simulink model "ZT_VehCtrl_18B_CAN"  (R2018b)
settings: Solver=FixedStepAuto  StartTime=0.0  StopTime=inf  FixedStep=0.005  RelTol=1e-3
InitFcn:
  | mbd_mpc_consistency_checks(bdroot(gcs));
values from neighbouring files (symbols this model uses):
  BatoverTempTh = single(80)    [VCU_INIT.m]
  BRS_PwrValid = single(5)    [VCU_INIT.m]
  BRSEnSpdTh1 = single(10)    [VCU_INIT.m]
  BRSEnSpdTh2 = single(20)    [VCU_INIT.m]
  MCUTempAlarmTh = single (60)    [VCU_INIT.m]
  mps2kmh = single(3.6)    [VCU_INIT.m]
  MtrPwrFac = single(1/9550)    [VCU_INIT.m]
  MtrTempAlarmTh = single (50)    [VCU_INIT.m]
  Padle1Signal1_Th = [PadleSignal1_min,PadleSignal1_max]    [VCU_INIT.m]
  Padle1Signal2_Th = [PadleSignal2_min,PadleSignal2_max]    [VCU_INIT.m]
  PadleSignal1_max = 3.84    [VCU_INIT.m]
  PadleSignal1_min = 0.75    [VCU_INIT.m]
  PadleSignal2_max = 1.92    [VCU_INIT.m]
  PadleSignal2_min = 0.375    [VCU_INIT.m]
  PadleValid = 0.05    [VCU_INIT.m]
  PwrLimFactor = single(0.5)    [VCU_INIT.m]
  Ratio = single(1)    [VCU_INIT.m]
  rpm2mps = single(2*pi/60 * WhlRadius/Ratio)    [VCU_INIT.m]
  SOCLowTh = single(20)    [VCU_INIT.m]
  VehPwrBackwardMax = VehPwrMax * single(0.3)    [VCU_INIT.m]
  VehPwrMax = single(MtrPwrMax * 4)    [VCU_INIT.m]
  VehTrqBackwardMax = VehTrqMax * single(0.3)    [VCU_INIT.m]
  VehTrqMax = single(MtrTrqMax * Ratio *4)    [VCU_INIT.m]
  WhlRadius = single(1)    [VCU_INIT.m]
undefined symbols (not defined in the file or in its folder): Delay_Charge, Delay_Discharge, fifo_0_vect, fifo_1_vect, LQFP, pts1_fifo_0_vect, pts1_fifo_1_vect, pts2_fifo_0_vect, pts2_fifo_1_vect, pts3_fifo_0_vect, pts3_fifo_1_vect, pts4_fifo_0_vect, pts4_fifo_1_vect
libraries: mbd_mpc574x_ec_toolbox x157, canmsglib x74, simulink x38
(part 10 of 12)

== system ZT_VehCtrl_18B_CAN/SigIn/CAN1/HVC4_RlySt/UNPACK ==
  ID : Inport
  data : Inport  Port=2
  length : Inport  Port=3
  timestamp : Inport  Port=4
  Action Port : ActionPort  ActionType=case
  Add : Sum
  Bus Creator : BusCreator  Inputs=7  OutDataTypeStr=Bus: CAN_MESSAGE_BUS  NonVirtualBus=on
  Bus Creator1 : BusCreator  Inputs=13
  CAN Unpack6 : canmsglib/CAN Unpack  CANdbFile=D:\VCU\VCU_SL_ZhengZhou\ZT2\模型与接口\CAN_DBC\动力CANB_GBK.dbc  MsgList=(none)  MsgName=HVC4_RlySt  MsgIDType=Extended (29-bit identifier)  MsgIdentifier=402916769  MsgLength=8  SignalInfo=HVC4_Life$60$4$1$2$1$0$1$0$0$15$#HVC_FaultCode$24$32$1$2$1$0$1$0$0$4294967295$#HVC_FaultLevel$56$2$1$2$1$0$1$0$0$3$#KM01_MotDrv1MainSt$0$2$1$2$1$0$1$0$0$3$#KM02_MotDrv2MainSt$4$2$1$2$1$0$1$0$0$3$#KM03_PaxACSt$8$2$1$2$1$0$1$0$0$3$#KM04_MotDrv1PreSt$2$2$1$2$1$0$1$0$0$3$#KM05_MotDrv2PreSt$6$2$1$2$1$0$1$0$0$3$#KM06_PTCSt$10$2$1$2$1$0$1$0$0$3$#MotDrv1_PowOnSt$16$1$1$2$1$0$1$0$0$1$#MotDrv2_PowOnSt$17$1$1$2$1$0$1$0$0$1$#PTC_PowOnSt$19$1$1$2$1$0$1$0$0$1$#PaxAC_PowOnSt$18$1$1$2$1$0$1$0$0$1$#  NSignals=13  IDPort=off  TimestampPort=off  ErrorPort=off  RemotePort=off  LengthPort=off  StatusPort=off  StartBits=str2num('[int32(60);int32(24);int32(56);int32(0);int32(4);int32(8);int32(2);int32(6);int32(10);int32(16);int32(17);int32(19);int32(18)]')  SignalSizes=str2num('[int32(4);int32(32);int32(2);int32(2);int32(2);int32(2);int32(2);int32(2);int32(2);int32(1);int32(1);int32(1);int32(1)]')  ByteOrders=str2num('[int32(1);int32(1);int32(1);int32(1);int32(1);int32(1);int32(1);int32(1);int32(1);int32(1);int32(1);int32(1);int32(1)]')  DataTypes=str2num('[int32(2);int32(2);int32(2);int32(2);int32(2);int32(2);int32(2);int32(2);int32(2);int32(2);int32(2);int32(2);int32(2)]')  MultiplexTypes=str2num('[int32(1);int32(1);int32(1);int32(1);int32(1);int32(1);int32(1);int32(1);int32(1);int32(1);int32(1);int32(1);int32(1)]')  MultiplexValues=str2num('[double(0);double(0);double(0);double(0);double(0);double(0);double(0);double(0);double(0);double(0);double(0);double(0);double(0)]')  Factors=str2num('[double(1);double(1);double(1);double(1);double(1);double(1);double(1);double(1);double(1);double(1);double(1);double(1);double(1)]')  Offsets=str2num('[double(0);double(0);double(0);double(0);double(0);double(0);double(0);double(0);double(0);double(0);double(0);double(0);double(0)]')  Minimums=str2num('[double(0);double(0);double(0);double(0);double(0);double(0);double(0);double(0);double(0);double(0);double(0);double(0);double(0)]')  Maximums=str2num('[double(15);double(4294967295);double(3);double(3);double(3);double(3);double(3);double(3);double(3);double(1);double(1);double(1);double(1)]')  ApplyMinMax=off
      settings: SourceProductName=Simulink Real-Time  SourceProductBaseCode=XP  DataFormat=CANdb specified signals
  Constant : Constant  OutDataTypeStr=uint8
  Constant1 : Constant  OutDataTypeStr=uint8
  Constant4 : Constant  Value=0  OutDataTypeStr=uint8
  Constant5 : Constant  Value=0  OutDataTypeStr=uint8
  Data Store Read : DataStoreRead  DataStoreName=Cnt_HVC4
  Data Store Write : DataStoreWrite  DataStoreName=Cnt_HVC4
  Data Type Conversion{,14..15,17} (4 alike) : DataTypeConversion  OutDataTypeStr=uint8
  Data Type Conversion{1..4} (4 alike) : DataTypeConversion  OutDataTypeStr=boolean
  Data Type Conversion{5..13} (9 alike) : DataTypeConversion  OutDataTypeStr=single
  Data Type Conversion18 : DataTypeConversion  OutDataTypeStr=uint32
  Data Type Conversion19 : DataTypeConversion  OutDataTypeStr=double
  Message : Outport
  wires:
  Constant4/1 -> Data Type Conversion15/1
  length/1 -> Data Type Conversion14/1
  data/1 -> Bus Creator/7  "Data"
  Data Type Conversion18/1 -> Bus Creator/5  "ID"
  Constant1/1 -> Data Type Conversion/1
  Constant5/1 -> Data Type Conversion17/1
  ID/1 -> Data Type Conversion18/1
  Data Type Conversion19/1 -> Bus Creator/6  "Timestamp"
  timestamp/1 -> Data Type Conversion19/1
  Data Type Conversion17/1 -> Bus Creator/4  "Error"
  Bus Creator/1 -> CAN Unpack6/1  "CAN_Msg_In"
  Data Type Conversion/1 -> Bus Creator/1  "Extended"
  Data Type Conversion14/1 -> Bus Creator/2  "Length"
  Data Type Conversion15/1 -> Bus Creator/3  "Remote"
  Bus Creator1/1 -> Message/1
  CAN Unpack6/6 -> Data Type Conversion8/1
  CAN Unpack6/5 -> Data Type Conversion9/1
  CAN Unpack6/7 -> Data Type Conversion7/1
  CAN Unpack6/4 -> Data Type Conversion10/1
  CAN Unpack6/8 -> Data Type Conversion6/1
  CAN Unpack6/3 -> Data Type Conversion11/1
  CAN Unpack6/9 -> Data Type Conversion5/1
  CAN Unpack6/2 -> Data Type Conversion12/1
  CAN Unpack6/10 -> Data Type Conversion4/1
  CAN Unpack6/1 -> Data Type Conversion13/1
  CAN Unpack6/11 -> Data Type Conversion3/1
  CAN Unpack6/12 -> Data Type Conversion2/1
  CAN Unpack6/13 -> Data Type Conversion1/1
  Data Type Conversion1/1 -> Bus Creator1/13  "PaxAC_PowOnSt"
  Data Type Conversion2/1 -> Bus Creator1/12  "PTC_PowOnSt"
  Data Type Conversion3/1 -> Bus Creator1/11  "MotDrv2_PowOnSt"
  Data Type Conversion4/1 -> Bus Creator1/10  "MotDrv1_PowOnSt"
  Data Type Conversion5/1 -> Bus Creator1/9  "KM06_PTCACSt"
  Data Type Conversion6/1 -> Bus Creator1/8  "KM05_MotDrv2PreSt"
  Data Type Conversion7/1 -> Bus Creator1/7  "KM04_MotDrv1PreSt"
  Data Type Conversion8/1 -> Bus Creator1/6  "KM03_PaxACSt"
  Data Type Conversion9/1 -> Bus Creator1/5  "KM02_MotDrv2MainSt"
  Data Type Conversion10/1 -> Bus Creator1/4  "KM01_MotDrv1MainSt"
  Data Type Conversion11/1 -> Bus Creator1/3  "HVC_FaultLevel"
  Data Type Conversion12/1 -> Bus Creator1/2  "HVC_FaultCode"
  Data Type Conversion13/1 -> Bus Creator1/1  "HVC4_Life"
  Add/1 -> Data Store Write/1
  Constant/1 -> Add/2
  Data Store Read/1 -> Add/1

== system ZT_VehCtrl_18B_CAN/SigIn/CAN1/HVC7_HV1/UNPACK ==
  ID : Inport
  data : Inport  Port=2
  length : Inport  Port=3
  timestamp : Inport  Port=4
  Action Port : ActionPort  ActionType=case
  Add : Sum
  Bus Creator : BusCreator  Inputs=7  OutDataTypeStr=Bus: CAN_MESSAGE_BUS  NonVirtualBus=on
  Bus Creator1 : BusCreator  Inputs=6
  CAN Unpack6 : canmsglib/CAN Unpack  CANdbFile=D:\VCU\VCU_SL_ZhengZhou\ZT2\模型与接口\CAN_DBC\动力CANB_GBK.dbc  MsgList=(none)  MsgName=HVC7_HV1  MsgIDType=Extended (29-bit identifier)  MsgIdentifier=403113377  MsgLength=8  SignalInfo=HVC5_Life$60$4$1$2$1$0$1$0$0$15$#MotDrv1_Vol$24$12$1$2$1$0$5.000000e-01$-1024$-1024$1.023500e+03$#MotDrv2_Vol$36$12$1$2$1$0$5.000000e-01$-1024$-1024$1.023500e+03$#PTC_Vol$12$12$1$2$1$0$5.000000e-01$-1024$-1024$1.023500e+03$#PaxAC_Vol$48$12$1$2$1$0$5.000000e-01$-1024$-1024$1.023500e+03$#PwrPos_Vol$0$12$1$2$1$0$5.000000e-01$-1024$-1024$1.023500e+03$#  NSignals=6  IDPort=off  TimestampPort=off  ErrorPort=off  RemotePort=off  LengthPort=off  StatusPort=off  StartBits=str2num('[int32(60);int32(24);int32(36);int32(12);int32(48);int32(0)]')  SignalSizes=str2num('[int32(4);int32(12);int32(12);int32(12);int32(12);int32(12)]')  ByteOrders=str2num('[int32(1);int32(1);int32(1);int32(1);int32(1);int32(1)]')  DataTypes=str2num('[int32(2);int32(2);int32(2);int32(2);int32(2);int32(2)]')  MultiplexTypes=str2num('[int32(1);int32(1);int32(1);int32(1);int32(1);int32(1)]')  MultiplexValues=str2num('[double(0);double(0);double(0);double(0);double(0);double(0)]')  Factors=str2num('[double(1);double(5.000000e-01);double(5.000000e-01);double(5.000000e-01);double(5.000000e-01);double(5.000000e-01)]')  Offsets=str2num('[double(0);double(-1024);double(-1024);double(-1024);double(-1024);double(-1024)]')  Minimums=str2num('[double(0);double(-1024);double(-1024);double(-1024);double(-1024);double(-1024)]')  Maximums=str2num('[double(15);double(1.023500e+03);double(1.023500e+03);double(1.023500e+03);double(1.023500e+03);double(1.023500e+03)]')  ApplyMinMax=off
      settings: SourceProductName=Simulink Real-Time  SourceProductBaseCode=XP  DataFormat=CANdb specified signals
  Constant : Constant  OutDataTypeStr=uint8
  Constant1 : Constant  OutDataTypeStr=uint8
  Constant4 : Constant  Value=0  OutDataTypeStr=uint8
  Constant5 : Constant  Value=0  OutDataTypeStr=uint8
  Data Store Read : DataStoreRead  DataStoreName=Cnt_HVC7
  Data Store Write : DataStoreWrite  DataStoreName=Cnt_HVC7
  Data Type Conversion{,14..15,17} (4 alike) : DataTypeConversion  OutDataTypeStr=uint8
  Data Type Conversion{1..6} (6 alike) : DataTypeConversion  OutDataTypeStr=single
  Data Type Conversion18 : DataTypeConversion  OutDataTypeStr=uint32
  Data Type Conversion19 : DataTypeConversion  OutDataTypeStr=double
  Message : Outport
  wires:
  Bus Creator1/1 -> Message/1
  Data Type Conversion15/1 -> Bus Creator/3  "Remote"
  Data Type Conversion14/1 -> Bus Creator/2  "Length"
  Data Type Conversion/1 -> Bus Creator/1  "Extended"
  Bus Creator/1 -> CAN Unpack6/1  "CAN_Msg_In"
  Data Type Conversion17/1 -> Bus Creator/4  "Error"
  timestamp/1 -> Data Type Conversion19/1
  Data Type Conversion19/1 -> Bus Creator/6  "Timestamp"
  ID/1 -> Data Type Conversion18/1
  Constant5/1 -> Data Type Conversion17/1
  Constant1/1 -> Data Type Conversion/1
  Data Type Conversion18/1 -> Bus Creator/5  "ID"
  data/1 -> Bus Creator/7  "Data"
  length/1 -> Data Type Conversion14/1
  Constant4/1 -> Data Type Conversion15/1
  CAN Unpack6/1 -> Data Type Conversion6/1
  CAN Unpack6/2 -> Data Type Conversion5/1
  CAN Unpack6/3 -> Data Type Conversion4/1
  CAN Unpack6/4 -> Data Type Conversion3/1
  CAN Unpack6/5 -> Data Type Conversion2/1
  CAN Unpack6/6 -> Data Type Conversion1/1
  Data Type Conversion1/1 -> Bus Creator1/6  "PwrPos_Vol"
  Data Type Conversion2/1 -> Bus Creator1/5  "PaxAC_Vol"
  Data Type Conversion3/1 -> Bus Creator1/4  "PTC_Vol"
  Data Type Conversion4/1 -> Bus Creator1/3  "MotDrv2_Vol"
  Data Type Conversion5/1 -> Bus Creator1/2  "MotDrv1_Vol"
  Data Type Conversion6/1 -> Bus Creator1/1  "HVC5_Life"
  Add/1 -> Data Store Write/1
  Constant/1 -> Add/2
  Data Store Read/1 -> Add/1

== system ZT_VehCtrl_18B_CAN/SigIn/CAN1/ISG MCU STATUS 1/UNPACK ==
  ID : Inport
  data : Inport  Port=2
  length : Inport  Port=3
  timestamp : Inport  Port=4
  Action Port : ActionPort  ActionType=case
  Add : Sum
  Bus Creator : BusCreator  Inputs=7  OutDataTypeStr=Bus: CAN_MESSAGE_BUS  NonVirtualBus=on
  Bus Creator1 : BusCreator  Inputs=7
  CAN Unpack6 : canmsglib/CAN Unpack  CANdbFile=D:\VCU\VCU_SL_ZhengZhou\ZT2\模型与接口\CAN_DBC\动力CANB_GBK.dbc  MsgList=(none)  MsgName=ISG_MCU_STATUS_1  MsgIDType=Extended (29-bit identifier)  MsgIdentifier=218038278  MsgLength=8  SignalInfo=Active_Discharge_Enable_Feedback$53$1$1$2$1$0$1$0$-Inf$Inf$#IGBT_Enable_Feedback$54$1$1$2$1$0$1$0$-Inf$Inf$#Life_counter$60$4$1$2$1$0$1$0$-Inf$Inf$#Motor_AC_Current$32$16$1$2$1$0$1.000000e-01$0$0$1000$#Motor_Speed$0$16$1$2$1$0$1$-15000$-15000$15000$#Motor_Torque$16$16$1$2$1$0$1$-5000$-5000$5000$#Precharge_Allow$52$1$1$2$1$0$1$0$-Inf$Inf$#  NSignals=7  IDPort=off  TimestampPort=off  ErrorPort=off  RemotePort=off  LengthPort=off  StatusPort=off  StartBits=str2num('[int32(53);int32(54);int32(60);int32(32);int32(0);int32(16);int32(52)]')  SignalSizes=str2num('[int32(1);int32(1);int32(4);int32(16);int32(16);int32(16);int32(1)]')  ByteOrders=str2num('[int32(1);int32(1);int32(1);int32(1);int32(1);int32(1);int32(1)]')  DataTypes=str2num('[int32(2);int32(2);int32(2);int32(2);int32(2);int32(2);int32(2)]')  MultiplexTypes=str2num('[int32(1);int32(1);int32(1);int32(1);int32(1);int32(1);int32(1)]')  MultiplexValues=str2num('[double(0);double(0);double(0);double(0);double(0);double(0);double(0)]')  Factors=str2num('[double(1);double(1);double(1);double(1.000000e-01);double(1);double(1);double(1)]')  Offsets=str2num('[double(0);double(0);double(0);double(0);double(-15000);double(-5000);double(0)]')  Minimums=str2num('[double(-Inf);double(-Inf);double(-Inf);double(0);double(-15000);double(-5000);double(-Inf)]')  Maximums=str2num('[double(Inf);double(Inf);double(Inf);double(1000);double(15000);double(5000);double(Inf)]')  ApplyMinMax=off
      settings: SourceProductName=Simulink Real-Time  SourceProductBaseCode=XP  DataFormat=CANdb specified signals
  Constant : Constant  OutDataTypeStr=uint8
  Constant1 : Constant  OutDataTypeStr=uint8
  Constant4 : Constant  Value=0  OutDataTypeStr=uint8
  Constant5 : Constant  Value=0  OutDataTypeStr=uint8
  Data Store Read : DataStoreRead  DataStoreName=Cnt_ISG1
  Data Store Write : DataStoreWrite  DataStoreName=Cnt_ISG1
  Data Type Conversion{,14..15,17} (4 alike) : DataTypeConversion  OutDataTypeStr=uint8
  Data Type Conversion1 : DataTypeConversion  OutDataTypeStr=boolean
  Data Type Conversion18 : DataTypeConversion  OutDataTypeStr=uint32
  Data Type Conversion19 : DataTypeConversion  OutDataTypeStr=double
  Data Type Conversion2 : DataTypeConversion  OutDataTypeStr=boolean
  Data Type Conversion{3..6} (4 alike) : DataTypeConversion  OutDataTypeStr=single
  Data Type Conversion7 : DataTypeConversion  OutDataTypeStr=boolean
  "Message " : Outport
  wires:
  Constant4/1 -> Data Type Conversion15/1
  length/1 -> Data Type Conversion14/1
  data/1 -> Bus Creator/7  "Data"
  Data Type Conversion18/1 -> Bus Creator/5  "ID"
  Constant1/1 -> Data Type Conversion/1
  Constant5/1 -> Data Type Conversion17/1
  ID/1 -> Data Type Conversion18/1
  Data Type Conversion19/1 -> Bus Creator/6  "Timestamp"
  timestamp/1 -> Data Type Conversion19/1
  Data Type Conversion17/1 -> Bus Creator/4  "Error"
  Bus Creator/1 -> CAN Unpack6/1  "CAN_Msg_In"
  Data Type Conversion/1 -> Bus Creator/1  "Extended"
  Data Type Conversion14/1 -> Bus Creator/2  "Length"
  Data Type Conversion15/1 -> Bus Creator/3  "Remote"
  CAN Unpack6/3 -> Data Type Conversion3/1
  CAN Unpack6/6 -> Data Type Conversion6/1
  CAN Unpack6/5 -> Data Type Conversion5/1
  CAN Unpack6/7 -> Data Type Conversion7/1
  CAN Unpack6/4 -> Data Type Conversion4/1
  Data Type Conversion3/1 -> Bus Creator1/3  "Life_counter"
  Data Type Conversion6/1 -> Bus Creator1/6  "Motor_Torque"
  CAN Unpack6/1 -> Data Type Conversion1/1
  Data Type Conversion4/1 -> Bus Creator1/4  "Motor_AC_Current"
  Data Type Conversion1/1 -> Bus Creator1/1  "Active_Discharge_Enable_Feedback"
  Data Type Conversion7/1 -> Bus Creator1/7  "Precharge_Allow"
  CAN Unpack6/2 -> Data Type Conversion2/1
  Data Type Conversion2/1 -> Bus Creator1/2  "IGBT_Enable_Feedback"
  Data Type Conversion5/1 -> Bus Creator1/5  "Motor_Speed"
  Bus Creator1/1 -> "Message "/1
  Constant/1 -> Add/2
  Data Store Read/1 -> Add/1
  Add/1 -> Data Store Write/1

== system ZT_VehCtrl_18B_CAN/SigIn/CAN1/ISG MCU STATUS 2/UNPACK ==
  ID : Inport
  data : Inport  Port=2
  length : Inport  Port=3
  timestamp : Inport  Port=4
  Action Port : ActionPort  ActionType=case
  Add : Sum
  Bus Creator : BusCreator  Inputs=7  OutDataTypeStr=Bus: CAN_MESSAGE_BUS  NonVirtualBus=on
  Bus Creator2 : BusCreator  Inputs=6
  CAN Unpack6 : canmsglib/CAN Unpack  CANdbFile=D:\VCU\VCU_SL_ZhengZhou\ZT2\模型与接口\CAN_DBC\动力CANB_GBK.dbc  MsgList=(none)  MsgName=ISG_MCU_STATUS2  MsgIDType=Extended (29-bit identifier)  MsgIdentifier=218038534  MsgLength=8  SignalInfo=Fail_Grade$48$4$1$2$1$0$1$0$-Inf$Inf$#Life_counter$60$4$1$2$1$0$1$0$-Inf$Inf$#MCU_temperature$8$8$1$2$1$0$1$-40$-40$215$#Motor_Temperature$0$8$1$2$1$0$1$-40$-40$215$#Torque_Limit_High$16$16$1$2$1$0$1$0$0$5000$#Torque_Limit_Low$32$16$1$2$1$0$1$-5000$-5000$0$#  NSignals=6  IDPort=off  TimestampPort=off  ErrorPort=off  RemotePort=off  LengthPort=off  StatusPort=off  StartBits=str2num('[int32(48);int32(60);int32(8);int32(0);int32(16);int32(32)]')  SignalSizes=str2num('[int32(4);int32(4);int32(8);int32(8);int32(16);int32(16)]')  ByteOrders=str2num('[int32(1);int32(1);int32(1);int32(1);int32(1);int32(1)]')  DataTypes=str2num('[int32(2);int32(2);int32(2);int32(2);int32(2);int32(2)]')  MultiplexTypes=str2num('[int32(1);int32(1);int32(1);int32(1);int32(1);int32(1)]')  MultiplexValues=str2num('[double(0);double(0);double(0);double(0);double(0);double(0)]')  Factors=str2num('[double(1);double(1);double(1);double(1);double(1);double(1)]')  Offsets=str2num('[double(0);double(0);double(-40);double(-40);double(0);double(-5000)]')  Minimums=str2num('[double(-Inf);double(-Inf);double(-40);double(-40);double(0);double(-5000)]')  Maximums=str2num('[double(Inf);double(Inf);double(215);double(215);double(5000);double(0)]')  ApplyMinMax=off
      settings: SourceProductName=Simulink Real-Time  SourceProductBaseCode=XP  DataFormat=CANdb specified signals
  Constant : Constant  OutDataTypeStr=uint8
  Constant1 : Constant  OutDataTypeStr=uint8
  Constant4 : Constant  Value=0  OutDataTypeStr=uint8
  Constant5 : Constant  Value=0  OutDataTypeStr=uint8
  Data Store Read : DataStoreRead  DataStoreName=Cnt_ISG2
  Data Store Write : DataStoreWrite  DataStoreName=Cnt_ISG2
  Data Type Conversion{,14..15,17} (4 alike) : DataTypeConversion  OutDataTypeStr=uint8
  Data Type Conversion{1..6} (6 alike) : DataTypeConversion  OutDataTypeStr=single
  Data Type Conversion18 : DataTypeConversion  OutDataTypeStr=uint32
  Data Type Conversion19 : DataTypeConversion  OutDataTypeStr=double
  Message1 : Outport
  wires:
  Data Type Conversion15/1 -> Bus Creator/3  "Remote"
  Data Type Conversion14/1 -> Bus Creator/2  "Length"
  Data Type Conversion/1 -> Bus Creator/1  "Extended"
  Bus Creator/1 -> CAN Unpack6/1  "CAN_Msg_In"
  Data Type Conversion17/1 -> Bus Creator/4  "Error"
  timestamp/1 -> Data Type Conversion19/1
  Data Type Conversion19/1 -> Bus Creator/6  "Timestamp"
  ID/1 -> Data Type Conversion18/1
  Constant5/1 -> Data Type Conversion17/1
  Constant1/1 -> Data Type Conversion/1
  Data Type Conversion18/1 -> Bus Creator/5  "ID"
  data/1 -> Bus Creator/7  "Data"
  length/1 -> Data Type Conversion14/1
  Constant4/1 -> Data Type Conversion15/1
  CAN Unpack6/6 -> Data Type Conversion6/1
  CAN Unpack6/1 -> Data Type Conversion1/1
  CAN Unpack6/2 -> Data Type Conversion2/1
  CAN Unpack6/5 -> Data Type Conversion5/1
  CAN Unpack6/4 -> Data Type Conversion4/1
  CAN Unpack6/3 -> Data Type Conversion3/1
  Data Type Conversion5/1 -> Bus Creator2/5  "Torque_Limit_High"
  Data Type Conversion6/1 -> Bus Creator2/6  "Torque_Limit_Low"
  Data Type Conversion4/1 -> Bus Creator2/4  "Motor_Temperature"
  Data Type Conversion2/1 -> Bus Creator2/2  "Life_counter"
  Data Type Conversion3/1 -> Bus Creator2/3  "MCU_temperature"
  Bus Creator2/1 -> Message1/1
  Data Type Conversion1/1 -> Bus Creator2/1  "Fail_Grade"
  Add/1 -> Data Store Write/1
  Data Store Read/1 -> Add/1
  Constant/1 -> Add/2

== system ZT_VehCtrl_18B_CAN/SigIn/CAN1/ISG MCU STATUS 3/UNPACK ==
  ID : Inport
  data : Inport  Port=2
  length : Inport  Port=3
  timestamp : Inport  Port=4
  Action Port : ActionPort  ActionType=case
  Add : Sum
  Bus Creator : BusCreator  Inputs=7  OutDataTypeStr=Bus: CAN_MESSAGE_BUS  NonVirtualBus=on
  Bus Creator1 : BusCreator  Inputs=5
  CAN Unpack6 : canmsglib/CAN Unpack  CANdbFile=D:\VCU\VCU_SL_ZhengZhou\ZT2\模型与接口\CAN_DBC\动力CANB_GBK.dbc  MsgList=(none)  MsgName=ISG_MCU_STATUS3  MsgIDType=Extended (29-bit identifier)  MsgIdentifier=218038790  MsgLength=8  SignalInfo=Alarm_Code$8$8$1$2$1$0$1$0$0$255$#DC_Current_A$16$16$1$2$1$0$1$-1000$-1000$1000$#DC_Voltage_V$32$16$1$2$1$0$1.000000e-01$0$0$1000$#Fault_Code$0$8$1$2$1$0$1$0$0$255$#Life_counter$48$4$1$2$1$0$1$0$0$15$#  NSignals=5  IDPort=off  TimestampPort=off  ErrorPort=off  RemotePort=off  LengthPort=off  StatusPort=off  StartBits=str2num('[int32(8);int32(16);int32(32);int32(0);int32(48)]')  SignalSizes=str2num('[int32(8);int32(16);int32(16);int32(8);int32(4)]')  ByteOrders=str2num('[int32(1);int32(1);int32(1);int32(1);int32(1)]')  DataTypes=str2num('[int32(2);int32(2);int32(2);int32(2);int32(2)]')  MultiplexTypes=str2num('[int32(1);int32(1);int32(1);int32(1);int32(1)]')  MultiplexValues=str2num('[double(0);double(0);double(0);double(0);double(0)]')  Factors=str2num('[double(1);double(1);double(1.000000e-01);double(1);double(1)]')  Offsets=str2num('[double(0);double(-1000);double(0);double(0);double(0)]')  Minimums=str2num('[double(0);double(-1000);double(0);double(0);double(0)]')  Maximums=str2num('[double(255);double(1000);double(1000);double(255);double(15)]')  ApplyMinMax=off
      settings: SourceProductName=Simulink Real-Time  SourceProductBaseCode=XP  DataFormat=CANdb specified signals
  Constant : Constant  OutDataTypeStr=uint8
  Constant1 : Constant  OutDataTypeStr=uint8
  Constant4 : Constant  Value=0  OutDataTypeStr=uint8
  Constant5 : Constant  Value=0  OutDataTypeStr=uint8
  Data Store Read : DataStoreRead  DataStoreName=Cnt_ISG3
  Data Store Write : DataStoreWrite  DataStoreName=Cnt_ISG3
  Data Type Conversion{,14..15,17} (4 alike) : DataTypeConversion  OutDataTypeStr=uint8
  Data Type Conversion{1..5} (5 alike) : DataTypeConversion  OutDataTypeStr=single
  Data Type Conversion18 : DataTypeConversion  OutDataTypeStr=uint32
  Data Type Conversion19 : DataTypeConversion  OutDataTypeStr=double
  Message : Outport
  wires:
  Constant4/1 -> Data Type Conversion15/1
  length/1 -> Data Type Conversion14/1
  data/1 -> Bus Creator/7  "Data"
  Data Type Conversion18/1 -> Bus Creator/5  "ID"
  Constant1/1 -> Data Type Conversion/1
  Constant5/1 -> Data Type Conversion17/1
  ID/1 -> Data Type Conversion18/1
  Data Type Conversion19/1 -> Bus Creator/6  "Timestamp"
  timestamp/1 -> Data Type Conversion19/1
  Data Type Conversion17/1 -> Bus Creator/4  "Error"
  Bus Creator/1 -> CAN Unpack6/1  "CAN_Msg_In"
  Data Type Conversion/1 -> Bus Creator/1  "Extended"
  Data Type Conversion14/1 -> Bus Creator/2  "Length"
  Data Type Conversion15/1 -> Bus Creator/3  "Remote"
  Data Type Conversion5/1 -> Bus Creator1/5  "Life_counter"
  Data Type Conversion3/1 -> Bus Creator1/3  "DC_Voltage_V"
  CAN Unpack6/2 -> Data Type Conversion2/1
  CAN Unpack6/4 -> Data Type Conversion4/1
  CAN Unpack6/1 -> Data Type Conversion1/1
  CAN Unpack6/3 -> Data Type Conversion3/1
  CAN Unpack6/5 -> Data Type Conversion5/1
  Data Type Conversion1/1 -> Bus Creator1/1  "Alarm_Code"
  Data Type Conversion2/1 -> Bus Creator1/2  "DC_Current_A"
  Data Type Conversion4/1 -> Bus Creator1/4  "Fault_Code"
  Bus Creator1/1 -> Message/1
  Add/1 -> Data Store Write/1
  Data Store Read/1 -> Add/1
  Constant/1 -> Add/2

== system ZT_VehCtrl_18B_CAN/SigIn/CAN1/MCU1Msg1/UNPACK ==
  ID : Inport
  data : Inport  Port=2
  length : Inport  Port=3
  timestamp : Inport  Port=4
  Action Port : ActionPort  ActionType=case
  Add : Sum
  Bus Creator : BusCreator  Inputs=7  OutDataTypeStr=Bus: CAN_MESSAGE_BUS  NonVirtualBus=on
  Bus Creator1 : BusCreator  Inputs=4
  CAN Unpack6 : canmsglib/CAN Unpack  CANdbFile=D:\VCU\VCU_SL_ZhengZhou\ZT2\模型与接口\CAN_DBC\动力CANB_GBK.dbc  MsgList=(none)  MsgName=MCU1Msg1  MsgIDType=Extended (29-bit identifier)  MsgIdentifier=406245615  MsgLength=8  SignalInfo=OilMotorBusCur$0$16$1$1$1$0$1.000000e-01$-600$-600$5.953500e+03$#OilMotorBusVolt$16$16$1$2$1$0$1$0$0$65535$#OilMotorSpd$32$16$1$1$1$0$1$-30000$-30000$35535$#OilMotorTrq$48$16$1$2$1$0$1.000000e-01$0$0$6.553500e+03$#  NSignals=4  IDPort=off  TimestampPort=off  ErrorPort=off  RemotePort=off  LengthPort=off  StatusPort=off  StartBits=str2num('[int32(0);int32(16);int32(32);int32(48)]')  SignalSizes=str2num('[int32(16);int32(16);int32(16);int32(16)]')  ByteOrders=str2num('[int32(1);int32(1);int32(1);int32(1)]')  DataTypes=str2num('[int32(1);int32(2);int32(1);int32(2)]')  MultiplexTypes=str2num('[int32(1);int32(1);int32(1);int32(1)]')  MultiplexValues=str2num('[double(0);double(0);double(0);double(0)]')  Factors=str2num('[double(1.000000e-01);double(1);double(1);double(1.000000e-01)]')  Offsets=str2num('[double(-600);double(0);double(-30000);double(0)]')  Minimums=str2num('[double(-600);double(0);double(-30000);double(0)]')  Maximums=str2num('[double(5.953500e+03);double(65535);double(35535);double(6.553500e+03)]')  ApplyMinMax=off
      settings: SourceProductName=Simulink Real-Time  SourceProductBaseCode=XP  DataFormat=CANdb specified signals
  Constant : Constant  OutDataTypeStr=uint8
  Constant1 : Constant  OutDataTypeStr=uint8
  Constant4 : Constant  Value=0  OutDataTypeStr=uint8
  Constant5 : Constant  Value=0  OutDataTypeStr=uint8
  Data Store Read : DataStoreRead  DataStoreName=Cnt_MCU1_1
  Data Store Write : DataStoreWrite  DataStoreName=Cnt_MCU1_1
  Data Type Conversion{,14..15,17} (4 alike) : DataTypeConversion  OutDataTypeStr=uint8
  Data Type Conversion{1..4} (4 alike) : DataTypeConversion  OutDataTypeStr=single
  Data Type Conversion18 : DataTypeConversion  OutDataTypeStr=uint32
  Data Type Conversion19 : DataTypeConversion  OutDataTypeStr=double
  Message : Outport
  wires:
  Bus Creator1/1 -> Message/1
  Data Type Conversion15/1 -> Bus Creator/3  "Remote"
  Data Type Conversion14/1 -> Bus Creator/2  "Length"
  Data Type Conversion/1 -> Bus Creator/1  "Extended"
  Bus Creator/1 -> CAN Unpack6/1  "CAN_Msg_In"
  Data Type Conversion17/1 -> Bus Creator/4  "Error"
  timestamp/1 -> Data Type Conversion19/1
  Data Type Conversion19/1 -> Bus Creator/6  "Timestamp"
  ID/1 -> Data Type Conversion18/1
  Constant5/1 -> Data Type Conversion17/1
  Constant1/1 -> Data Type Conversion/1
  Data Type Conversion18/1 -> Bus Creator/5  "ID"
  data/1 -> Bus Creator/7  "Data"
  length/1 -> Data Type Conversion14/1
  Constant4/1 -> Data Type Conversion15/1
  CAN Unpack6/1 -> Data Type Conversion1/1
  CAN Unpack6/2 -> Data Type Conversion2/1
  CAN Unpack6/3 -> Data Type Conversion3/1
  CAN Unpack6/4 -> Data Type Conversion4/1
  Data Type Conversion1/1 -> Bus Creator1/1  "OilMotorBusCur"
  Data Type Conversion2/1 -> Bus Creator1/2  "OilMotorBusVolt"
  Data Type Conversion3/1 -> Bus Creator1/3  "OilMotorSpd"
  Data Type Conversion4/1 -> Bus Creator1/4  "OilMotorTrq"
  Constant/1 -> Add/2
  Data Store Read/1 -> Add/1
  Add/1 -> Data Store Write/1

== system ZT_VehCtrl_18B_CAN/SigIn/CAN1/MCU1Msg2/UNPACK ==
  ID : Inport
  data : Inport  Port=2
  length : Inport  Port=3
  timestamp : Inport  Port=4
  Action Port : ActionPort  ActionType=case
  Add : Sum
  Bus Creator : BusCreator  Inputs=7  OutDataTypeStr=Bus: CAN_MESSAGE_BUS  NonVirtualBus=on
  Bus Creator1 : BusCreator  Inputs=9
  CAN Unpack6 : canmsglib/CAN Unpack  CANdbFile=D:\VCU\VCU_SL_ZhengZhou\ZT2\模型与接口\CAN_DBC\动力CANB_GBK.dbc  MsgList=(none)  MsgName=MCU1Msg2  MsgIDType=Extended (29-bit identifier)  MsgIdentifier=406311151  MsgLength=8  SignalInfo=OilMotorAntiSlipSt$7$1$1$2$1$0$1$0$0$1$#OilMotorBusCounter$56$8$1$2$1$0$1$0$0$255$#OilMotorFaultCode$24$8$1$2$1$0$1$0$0$100$#OilMotorFaultLevel$8$2$1$2$1$0$1$0$0$3$#OilMotorMCUID$32$16$1$2$1$0$1$0$0$65535$#OilMotorPwrLimitpct$16$8$1$2$1$0$1$0$0$100$#OilMotorSt$0$4$1$2$1$0$1$0$0$15$#OilMotorWorkModeSt$4$3$1$2$1$0$1$0$0$15$#Reserved$48$8$1$2$1$0$1$0$0$255$#  NSignals=9  IDPort=off  TimestampPort=off  ErrorPort=off  RemotePort=off  LengthPort=off  StatusPort=off  StartBits=str2num('[int32(7);int32(56);int32(24);int32(8);int32(32);int32(16);int32(0);int32(4);int32(48)]')  SignalSizes=str2num('[int32(1);int32(8);int32(8);int32(2);int32(16);int32(8);int32(4);int32(3);int32(8)]')  ByteOrders=str2num('[int32(1);int32(1);int32(1);int32(1);int32(1);int32(1);int32(1);int32(1);int32(1)]')  DataTypes=str2num('[int32(2);int32(2);int32(2);int32(2);int32(2);int32(2);int32(2);int32(2);int32(2)]')  MultiplexTypes=str2num('[int32(1);int32(1);int32(1);int32(1);int32(1);int32(1);int32(1);int32(1);int32(1)]')  MultiplexValues=str2num('[double(0);double(0);double(0);double(0);double(0);double(0);double(0);double(0);double(0)]')  Factors=str2num('[double(1);double(1);double(1);double(1);double(1);double(1);double(1);double(1);double(1)]')  Offsets=str2num('[double(0);double(0);double(0);double(0);double(0);double(0);double(0);double(0);double(0)]')  Minimums=str2num('[double(0);double(0);double(0);double(0);double(0);double(0);double(0);double(0);double(0)]')  Maximums=str2num('[double(1);double(255);double(100);double(3);double(65535);double(100);double(15);double(15);double(255)]')  ApplyMinMax=off
      settings: SourceProductName=Simulink Real-Time  SourceProductBaseCode=XP  DataFormat=CANdb specified signals
  Constant : Constant  OutDataTypeStr=uint8
  Constant1 : Constant  OutDataTypeStr=uint8
  Constant4 : Constant  Value=0  OutDataTypeStr=uint8
  Constant5 : Constant  Value=0  OutDataTypeStr=uint8
  Data Store Read : DataStoreRead  DataStoreName=Cnt_MCU1_2
  Data Store Write : DataStoreWrite  DataStoreName=Cnt_MCU1_2
  Data Type Conversion{,14..15,17} (4 alike) : DataTypeConversion  OutDataTypeStr=uint8
  Data Type Conversion1 : DataTypeConversion  OutDataTypeStr=boolean
  Data Type Conversion18 : DataTypeConversion  OutDataTypeStr=uint32
  Data Type Conversion19 : DataTypeConversion  OutDataTypeStr=double
  Data Type Conversion{2..9} (8 alike) : DataTypeConversion  OutDataTypeStr=single
  Message : Outport
  wires:
  Constant4/1 -> Data Type Conversion15/1
  length/1 -> Data Type Conversion14/1
  data/1 -> Bus Creator/7  "Data"
  Data Type Conversion18/1 -> Bus Creator/5  "ID"
  Constant1/1 -> Data Type Conversion/1
  Constant5/1 -> Data Type Conversion17/1
  ID/1 -> Data Type Conversion18/1
  Data Type Conversion19/1 -> Bus Creator/6  "Timestamp"
  timestamp/1 -> Data Type Conversion19/1
  Data Type Conversion17/1 -> Bus Creator/4  "Error"
  Bus Creator/1 -> CAN Unpack6/1  "CAN_Msg_In"
  Data Type Conversion/1 -> Bus Creator/1  "Extended"
  Data Type Conversion14/1 -> Bus Creator/2  "Length"
  Data Type Conversion15/1 -> Bus Creator/3  "Remote"
  Bus Creator1/1 -> Message/1
  CAN Unpack6/1 -> Data Type Conversion1/1
  CAN Unpack6/2 -> Data Type Conversion2/1
  CAN Unpack6/3 -> Data Type Conversion3/1
  CAN Unpack6/4 -> Data Type Conversion4/1
  CAN Unpack6/5 -> Data Type Conversion5/1
  CAN Unpack6/6 -> Data Type Conversion6/1
  CAN Unpack6/7 -> Data Type Conversion7/1
  CAN Unpack6/8 -> Data Type Conversion8/1
  CAN Unpack6/9 -> Data Type Conversion9/1
  Data Type Conversion1/1 -> Bus Creator1/1  "OilMotorAntiSlipSt"
  Data Type Conversion2/1 -> Bus Creator1/2  "OilMotorBusCounter"
  Data Type Conversion3/1 -> Bus Creator1/3  "OilMotorFaultCode"
  Data Type Conversion4/1 -> Bus Creator1/4  "OilMotorFaultLevel"
  Data Type Conversion5/1 -> Bus Creator1/5  "OilMotorMCUID"
  Data Type Conversion6/1 -> Bus Creator1/6  "OilMotorPwrLimitpct"
  Data Type Conversion7/1 -> Bus Creator1/7  "OilMotorSt"
  Data Type Conversion8/1 -> Bus Creator1/8  "OilMotorWorkModeSt"
  Data Type Conversion9/1 -> Bus Creator1/9  "Reserved"
  Data Store Read/1 -> Add/1
  Add/1 -> Data Store Write/1
  Constant/1 -> Add/2

== system ZT_VehCtrl_18B_CAN/SigIn/CAN1/MCU1Msg3/UNPACK ==
  ID : Inport
  data : Inport  Port=2
  length : Inport  Port=3
  timestamp : Inport  Port=4
  Action Port : ActionPort  ActionType=case
  Add : Sum
  Bus Creator : BusCreator  Inputs=7  OutDataTypeStr=Bus: CAN_MESSAGE_BUS  NonVirtualBus=on
  Bus Creator1 : BusCreator  Inputs=6
  CAN Unpack6 : canmsglib/CAN Unpack  CANdbFile=D:\VCU\VCU_SL_ZhengZhou\ZT2\模型与接口\CAN_DBC\动力CANB_GBK.dbc  MsgList=(none)  MsgName=MCU1Msg3  MsgIDType=Extended (29-bit identifier)  MsgIdentifier=406376687  MsgLength=8  SignalInfo=OilMotorMCUTemp1$24$8$1$1$1$0$1$-50$-50$205$#OilMotorMCUTemp2$32$8$1$1$1$0$1$-50$-50$205$#OilMotorMCUTemp3$40$8$1$1$1$0$1$-50$-50$205$#OilMotorTemp1$0$8$1$1$1$0$1$-50$-50$205$#OilMotorTemp2$8$8$1$1$1$0$1$-50$-50$205$#OilMotorTemp3$16$8$1$1$1$0$1$-50$-50$205$#  NSignals=6  IDPort=off  TimestampPort=off  ErrorPort=off  RemotePort=off  LengthPort=off  StatusPort=off  StartBits=str2num('[int32(24);int32(32);int32(40);int32(0);int32(8);int32(16)]')  SignalSizes=str2num('[int32(8);int32(8);int32(8);int32(8);int32(8);int32(8)]')  ByteOrders=str2num('[int32(1);int32(1);int32(1);int32(1);int32(1);int32(1)]')  DataTypes=str2num('[int32(1);int32(1);int32(1);int32(1);int32(1);int32(1)]')  MultiplexTypes=str2num('[int32(1);int32(1);int32(1);int32(1);int32(1);int32(1)]')  MultiplexValues=str2num('[double(0);double(0);double(0);double(0);double(0);double(0)]')  Factors=str2num('[double(1);double(1);double(1);double(1);double(1);double(1)]')  Offsets=str2num('[double(-50);double(-50);double(-50);double(-50);double(-50);double(-50)]')  Minimums=str2num('[double(-50);double(-50);double(-50);double(-50);double(-50);double(-50)]')  Maximums=str2num('[double(205);double(205);double(205);double(205);double(205);double(205)]')  ApplyMinMax=off
      settings: SourceProductName=Simulink Real-Time  SourceProductBaseCode=XP  DataFormat=CANdb specified signals
  Constant : Constant  OutDataTypeStr=uint8
  Constant1 : Constant  OutDataTypeStr=uint8
  Constant4 : Constant  Value=0  OutDataTypeStr=uint8
  Constant5 : Constant  Value=0  OutDataTypeStr=uint8
  Data Store Read : DataStoreRead  DataStoreName=Cnt_MCU1_3
  Data Store Write : DataStoreWrite  DataStoreName=Cnt_MCU1_3
  Data Type Conversion{,14..15,17} (4 alike) : DataTypeConversion  OutDataTypeStr=uint8
  Data Type Conversion{1..6} (6 alike) : DataTypeConversion  OutDataTypeStr=single
  Data Type Conversion18 : DataTypeConversion  OutDataTypeStr=uint32
  Data Type Conversion19 : DataTypeConversion  OutDataTypeStr=double
  Message : Outport
  wires:
  Bus Creator1/1 -> Message/1
  Data Type Conversion15/1 -> Bus Creator/3  "Remote"
  Data Type Conversion14/1 -> Bus Creator/2  "Length"
  Data Type Conversion/1 -> Bus Creator/1  "Extended"
  Bus Creator/1 -> CAN Unpack6/1  "CAN_Msg_In"
  Data Type Conversion17/1 -> Bus Creator/4  "Error"
  timestamp/1 -> Data Type Conversion19/1
  Data Type Conversion19/1 -> Bus Creator/6  "Timestamp"
  ID/1 -> Data Type Conversion18/1
  Constant5/1 -> Data Type Conversion17/1
  Constant1/1 -> Data Type Conversion/1
  Data Type Conversion18/1 -> Bus Creator/5  "ID"
  data/1 -> Bus Creator/7  "Data"
  length/1 -> Data Type Conversion14/1
  Constant4/1 -> Data Type Conversion15/1
  CAN Unpack6/1 -> Data Type Conversion1/1
  CAN Unpack6/2 -> Data Type Conversion2/1
  CAN Unpack6/3 -> Data Type Conversion3/1
  CAN Unpack6/4 -> Data Type Conversion4/1
  CAN Unpack6/5 -> Data Type Conversion5/1
  CAN Unpack6/6 -> Data Type Conversion6/1
  Data Type Conversion1/1 -> Bus Creator1/1  "OilMotorMCUTemp1"
  Data Type Conversion2/1 -> Bus Creator1/2  "OilMotorMCUTemp2"
  Data Type Conversion3/1 -> Bus Creator1/3  "OilMotorMCUTemp3"
  Data Type Conversion4/1 -> Bus Creator1/4  "OilMotorTemp1"
  Data Type Conversion5/1 -> Bus Creator1/5  "OilMotorTemp2"
  Data Type Conversion6/1 -> Bus Creator1/6  "OilMotorTemp3"
  Data Store Read/1 -> Add/1
  Add/1 -> Data Store Write/1
  Constant/1 -> Add/2

== system ZT_VehCtrl_18B_CAN/SigIn/CAN1/MCU2Msg1/UNPACK ==
  ID : Inport
  data : Inport  Port=2
  length : Inport  Port=3
  timestamp : Inport  Port=4
  Action Port : ActionPort  ActionType=case
  Add : Sum
  Bus Creator : BusCreator  Inputs=7  OutDataTypeStr=Bus: CAN_MESSAGE_BUS  NonVirtualBus=on
  Bus Creator1 : BusCreator  Inputs=4
  CAN Unpack6 : canmsglib/CAN Unpack  CANdbFile=D:\VCU\VCU_SL_ZhengZhou\ZT2\模型与接口\CAN_DBC\动力CANB_GBK.dbc  MsgList=(none)  MsgName=MCU2Msg1  MsgIDType=Extended (29-bit identifier)  MsgIdentifier=406245617  MsgLength=8  SignalInfo=DrvMotorBusCur$0$16$1$1$1$0$1.000000e-01$-600$-600$5.953500e+03$#DrvMotorBusVolt$16$16$1$2$1$0$1$0$0$65535$#DrvMotorSpd$32$16$1$1$1$0$1$-30000$-30000$35535$#DrvMotorTrq$48$16$1$2$1$0$1.000000e-01$0$0$6.553500e+03$#  NSignals=4  IDPort=off  TimestampPort=off  ErrorPort=off  RemotePort=off  LengthPort=off  StatusPort=off  StartBits=str2num('[int32(0);int32(16);int32(32);int32(48)]')  SignalSizes=str2num('[int32(16);int32(16);int32(16);int32(16)]')  ByteOrders=str2num('[int32(1);int32(1);int32(1);int32(1)]')  DataTypes=str2num('[int32(1);int32(2);int32(1);int32(2)]')  MultiplexTypes=str2num('[int32(1);int32(1);int32(1);int32(1)]')  MultiplexValues=str2num('[double(0);double(0);double(0);double(0)]')  Factors=str2num('[double(1.000000e-01);double(1);double(1);double(1.000000e-01)]')  Offsets=str2num('[double(-600);double(0);double(-30000);double(0)]')  Minimums=str2num('[double(-600);double(0);double(-30000);double(0)]')  Maximums=str2num('[double(5.953500e+03);double(65535);double(35535);double(6.553500e+03)]')  ApplyMinMax=off
      settings: SourceProductName=Simulink Real-Time  SourceProductBaseCode=XP  DataFormat=CANdb specified signals
  Constant : Constant  OutDataTypeStr=uint8
  Constant1 : Constant  OutDataTypeStr=uint8
  Constant4 : Constant  Value=0  OutDataTypeStr=uint8
  Constant5 : Constant  Value=0  OutDataTypeStr=uint8
  Data Store Read : DataStoreRead  DataStoreName=Cnt_MCU2_1
  Data Store Write : DataStoreWrite  DataStoreName=Cnt_MCU2_1
  Data Type Conversion{,14..15,17} (4 alike) : DataTypeConversion  OutDataTypeStr=uint8
  Data Type Conversion{1..4} (4 alike) : DataTypeConversion  OutDataTypeStr=single
  Data Type Conversion18 : DataTypeConversion  OutDataTypeStr=uint32
  Data Type Conversion19 : DataTypeConversion  OutDataTypeStr=double
  Message : Outport
  wires:
  Constant4/1 -> Data Type Conversion15/1
  length/1 -> Data Type Conversion14/1
  data/1 -> Bus Creator/7  "Data"
  Data Type Conversion18/1 -> Bus Creator/5  "ID"
  Constant1/1 -> Data Type Conversion/1
  Constant5/1 -> Data Type Conversion17/1
  ID/1 -> Data Type Conversion18/1
  Data Type Conversion19/1 -> Bus Creator/6  "Timestamp"
  timestamp/1 -> Data Type Conversion19/1
  Data Type Conversion17/1 -> Bus Creator/4  "Error"
  Bus Creator/1 -> CAN Unpack6/1  "CAN_Msg_In"
  Data Type Conversion/1 -> Bus Creator/1  "Extended"
  Data Type Conversion14/1 -> Bus Creator/2  "Length"
  Data Type Conversion15/1 -> Bus Creator/3  "Remote"
  Bus Creator1/1 -> Message/1
  CAN Unpack6/1 -> Data Type Conversion1/1
  CAN Unpack6/2 -> Data Type Conversion2/1
  CAN Unpack6/3 -> Data Type Conversion3/1
  CAN Unpack6/4 -> Data Type Conversion4/1
  Data Type Conversion1/1 -> Bus Creator1/1  "DrvMotorBusCur"
  Data Type Conversion2/1 -> Bus Creator1/2  "DrvMotorBusVolt"
  Data Type Conversion3/1 -> Bus Creator1/3  "DrvMotorSpd"
  Data Type Conversion4/1 -> Bus Creator1/4  "DrvMotorTrq"
  Data Store Read/1 -> Add/1
  Add/1 -> Data Store Write/1
  Constant/1 -> Add/2

== system ZT_VehCtrl_18B_CAN/SigIn/CAN1/MCU2Msg2/UNPACK ==
  ID : Inport
  data : Inport  Port=2
  length : Inport  Port=3
  timestamp : Inport  Port=4
  Action Port : ActionPort  ActionType=case
  Add : Sum
  Bus Creator : BusCreator  Inputs=7  OutDataTypeStr=Bus: CAN_MESSAGE_BUS  NonVirtualBus=on
  Bus Creator1 : BusCreator  Inputs=9
  CAN Unpack6 : canmsglib/CAN Unpack  CANdbFile=D:\VCU\VCU_SL_ZhengZhou\ZT2\模型与接口\CAN_DBC\动力CANB_GBK.dbc  MsgList=(none)  MsgName=MCU2Msg2  MsgIDType=Extended (29-bit identifier)  MsgIdentifier=406311153  MsgLength=8  SignalInfo=DrvMotorAntiSlipSt$7$1$1$2$1$0$1$0$0$1$#DrvMotorBusCounter$56$8$1$2$1$0$1$0$0$255$#DrvMotorFaultCode$24$8$1$2$1$0$1$0$0$100$#DrvMotorFaultLevel$8$2$1$2$1$0$1$0$0$3$#DrvMotorMCUID$32$16$1$2$1$0$1$0$0$65535$#DrvMotorPwrLimitpct$16$8$1$2$1$0$1$0$0$100$#DrvMotorSt$0$4$1$2$1$0$1$0$0$15$#DrvMotorWorkModeSt$4$3$1$2$1$0$1$0$0$15$#Reserved$48$8$1$2$1$0$1$0$0$255$#  NSignals=9  IDPort=off  TimestampPort=off  ErrorPort=off  RemotePort=off  LengthPort=off  StatusPort=off  StartBits=str2num('[int32(7);int32(56);int32(24);int32(8);int32(32);int32(16);int32(0);int32(4);int32(48)]')  SignalSizes=str2num('[int32(1);int32(8);int32(8);int32(2);int32(16);int32(8);int32(4);int32(3);int32(8)]')  ByteOrders=str2num('[int32(1);int32(1);int32(1);int32(1);int32(1);int32(1);int32(1);int32(1);int32(1)]')  DataTypes=str2num('[int32(2);int32(2);int32(2);int32(2);int32(2);int32(2);int32(2);int32(2);int32(2)]')  MultiplexTypes=str2num('[int32(1);int32(1);int32(1);int32(1);int32(1);int32(1);int32(1);int32(1);int32(1)]')  MultiplexValues=str2num('[double(0);double(0);double(0);double(0);double(0);double(0);double(0);double(0);double(0)]')  Factors=str2num('[double(1);double(1);double(1);double(1);double(1);double(1);double(1);double(1);double(1)]')  Offsets=str2num('[double(0);double(0);double(0);double(0);double(0);double(0);double(0);double(0);double(0)]')  Minimums=str2num('[double(0);double(0);double(0);double(0);double(0);double(0);double(0);double(0);double(0)]')  Maximums=str2num('[double(1);double(255);double(100);double(3);double(65535);double(100);double(15);double(15);double(255)]')  ApplyMinMax=off
      settings: SourceProductName=Simulink Real-Time  SourceProductBaseCode=XP  DataFormat=CANdb specified signals
  Constant : Constant  OutDataTypeStr=uint8
  Constant1 : Constant  OutDataTypeStr=uint8
  Constant4 : Constant  Value=0  OutDataTypeStr=uint8
  Constant5 : Constant  Value=0  OutDataTypeStr=uint8
  Data Store Read : DataStoreRead  DataStoreName=Cnt_MCU2_2
  Data Store Write : DataStoreWrite  DataStoreName=Cnt_MCU2_2
  Data Type Conversion{,14..15,17} (4 alike) : DataTypeConversion  OutDataTypeStr=uint8
  Data Type Conversion1 : DataTypeConversion  OutDataTypeStr=boolean
  Data Type Conversion18 : DataTypeConversion  OutDataTypeStr=uint32
  Data Type Conversion19 : DataTypeConversion  OutDataTypeStr=double
  Data Type Conversion{2..9} (8 alike) : DataTypeConversion  OutDataTypeStr=single
  Message : Outport
  wires:
  Bus Creator1/1 -> Message/1
  Data Type Conversion15/1 -> Bus Creator/3  "Remote"
  Data Type Conversion14/1 -> Bus Creator/2  "Length"
  Data Type Conversion/1 -> Bus Creator/1  "Extended"
  Bus Creator/1 -> CAN Unpack6/1  "CAN_Msg_In"
  Data Type Conversion17/1 -> Bus Creator/4  "Error"
  timestamp/1 -> Data Type Conversion19/1
  Data Type Conversion19/1 -> Bus Creator/6  "Timestamp"
  ID/1 -> Data Type Conversion18/1
  Constant5/1 -> Data Type Conversion17/1
  Constant1/1 -> Data Type Conversion/1
  Data Type Conversion18/1 -> Bus Creator/5  "ID"
  data/1 -> Bus Creator/7  "Data"
  length/1 -> Data Type Conversion14/1
  Constant4/1 -> Data Type Conversion15/1
  CAN Unpack6/1 -> Data Type Conversion1/1
  CAN Unpack6/2 -> Data Type Conversion3/1
  CAN Unpack6/3 -> Data Type Conversion2/1
  CAN Unpack6/4 -> Data Type Conversion4/1
  CAN Unpack6/5 -> Data Type Conversion5/1
  CAN Unpack6/6 -> Data Type Conversion6/1
  CAN Unpack6/7 -> Data Type Conversion7/1
  CAN Unpack6/8 -> Data Type Conversion8/1
  CAN Unpack6/9 -> Data Type Conversion9/1
  Data Type Conversion1/1 -> Bus Creator1/1  "DrvMotorAntiSlipSt"
  Data Type Conversion3/1 -> Bus Creator1/2  "DrvMotorBusCounter"
  Data Type Conversion2/1 -> Bus Creator1/3  "DrvMotorFaultCode"
  Data Type Conversion4/1 -> Bus Creator1/4  "DrvMotorFaultLevel"
  Data Type Conversion5/1 -> Bus Creator1/5  "DrvMotorMCUID"
  Data Type Conversion6/1 -> Bus Creator1/6  "DrvMotorPwrLimitpct"
  Data Type Conversion7/1 -> Bus Creator1/7  "DrvMotorSt"
  Data Type Conversion8/1 -> Bus Creator1/8  "DrvMotorWorkModeSt"
  Data Type Conversion9/1 -> Bus Creator1/9  "Reserved"
  Data Store Read/1 -> Add/1
  Add/1 -> Data Store Write/1
  Constant/1 -> Add/2

== system ZT_VehCtrl_18B_CAN/SigIn/CAN1/MCU2Msg3/UNPACK ==
  ID : Inport
  data : Inport  Port=2
  length : Inport  Port=3
  timestamp : Inport  Port=4
  Action Port : ActionPort  ActionType=case
  Add : Sum
  Bus Creator : BusCreator  Inputs=7  OutDataTypeStr=Bus: CAN_MESSAGE_BUS  NonVirtualBus=on
  Bus Creator1 : BusCreator  Inputs=6
  CAN Unpack6 : canmsglib/CAN Unpack  CANdbFile=D:\VCU\VCU_SL_ZhengZhou\ZT2\模型与接口\CAN_DBC\动力CANB_GBK.dbc  MsgList=(none)  MsgName=MCU2Msg3  MsgIDType=Extended (29-bit identifier)  MsgIdentifier=406376689  MsgLength=8  SignalInfo=DrvMotorMCUTemp1$24$8$1$1$1$0$1$-50$-50$205$#DrvMotorMCUTemp2$32$8$1$1$1$0$1$-50$-50$205$#DrvMotorMCUTemp3$40$8$1$1$1$0$1$-50$-50$205$#DrvMotorTemp1$0$8$1$1$1$0$1$-50$-50$205$#DrvMotorTemp2$8$8$1$1$1$0$1$-50$-50$205$#DrvMotorTemp3$16$8$1$1$1$0$1$-50$-50$205$#  NSignals=6  IDPort=off  TimestampPort=off  ErrorPort=off  RemotePort=off  LengthPort=off  StatusPort=off  StartBits=str2num('[int32(24);int32(32);int32(40);int32(0);int32(8);int32(16)]')  SignalSizes=str2num('[int32(8);int32(8);int32(8);int32(8);int32(8);int32(8)]')  ByteOrders=str2num('[int32(1);int32(1);int32(1);int32(1);int32(1);int32(1)]')  DataTypes=str2num('[int32(1);int32(1);int32(1);int32(1);int32(1);int32(1)]')  MultiplexTypes=str2num('[int32(1);int32(1);int32(1);int32(1);int32(1);int32(1)]')  MultiplexValues=str2num('[double(0);double(0);double(0);double(0);double(0);double(0)]')  Factors=str2num('[double(1);double(1);double(1);double(1);double(1);double(1)]')  Offsets=str2num('[double(-50);double(-50);double(-50);double(-50);double(-50);double(-50)]')  Minimums=str2num('[double(-50);double(-50);double(-50);double(-50);double(-50);double(-50)]')  Maximums=str2num('[double(205);double(205);double(205);double(205);double(205);double(205)]')  ApplyMinMax=off
      settings: SourceProductName=Simulink Real-Time  SourceProductBaseCode=XP  DataFormat=CANdb specified signals
  Constant : Constant  OutDataTypeStr=uint8
  Constant1 : Constant  OutDataTypeStr=uint8
  Constant4 : Constant  Value=0  OutDataTypeStr=uint8
  Constant5 : Constant  Value=0  OutDataTypeStr=uint8
  Data Store Read : DataStoreRead  DataStoreName=Cnt_MCU2_3
  Data Store Write : DataStoreWrite  DataStoreName=Cnt_MCU2_3
  Data Type Conversion{,14..15,17} (4 alike) : DataTypeConversion  OutDataTypeStr=uint8
  Data Type Conversion{1..6} (6 alike) : DataTypeConversion  OutDataTypeStr=single
  Data Type Conversion18 : DataTypeConversion  OutDataTypeStr=uint32
  Data Type Conversion19 : DataTypeConversion  OutDataTypeStr=double
  Message : Outport
  wires:
  Constant4/1 -> Data Type Conversion15/1
  length/1 -> Data Type Conversion14/1
  data/1 -> Bus Creator/7  "Data"
  Data Type Conversion18/1 -> Bus Creator/5  "ID"
  Constant1/1 -> Data Type Conversion/1
  Constant5/1 -> Data Type Conversion17/1
  ID/1 -> Data Type Conversion18/1
  Data Type Conversion19/1 -> Bus Creator/6  "Timestamp"
  timestamp/1 -> Data Type Conversion19/1
  Data Type Conversion17/1 -> Bus Creator/4  "Error"
  Bus Creator/1 -> CAN Unpack6/1  "CAN_Msg_In"
  Data Type Conversion/1 -> Bus Creator/1  "Extended"
  Data Type Conversion14/1 -> Bus Creator/2  "Length"
  Data Type Conversion15/1 -> Bus Creator/3  "Remote"
  Bus Creator1/1 -> Message/1
  CAN Unpack6/1 -> Data Type Conversion1/1
  CAN Unpack6/2 -> Data Type Conversion2/1
  CAN Unpack6/3 -> Data Type Conversion3/1
  CAN Unpack6/4 -> Data Type Conversion4/1
  CAN Unpack6/5 -> Data Type Conversion5/1
  CAN Unpack6/6 -> Data Type Conversion6/1
  Data Type Conversion1/1 -> Bus Creator1/1  "DrvMotorMCUTemp1"
  Data Type Conversion2/1 -> Bus Creator1/2  "DrvMotorMCUTemp2"
  Data Type Conversion3/1 -> Bus Creator1/3  "DrvMotorMCUTemp3"
  Data Type Conversion4/1 -> Bus Creator1/4  "DrvMotorTemp1"
  Data Type Conversion5/1 -> Bus Creator1/5  "DrvMotorTemp2"
  Data Type Conversion6/1 -> Bus Creator1/6  "DrvMotorTemp3"
  Data Store Read/1 -> Add/1
  Add/1 -> Data Store Write/1
  Constant/1 -> Add/2
